simulink model "roll_model_TRUCKSIM_18DOF_REVISED"  (R2023b)
settings: Solver=FixedStepAuto  StartTime=0.0  StopTime=20  FixedStep=0.0005  RelTol=1e-3
StopFcn:
  | save_dataset_18state;
libraries: Solver_SF x1
(part 3 of 5)

== matlab function roll_model_TRUCKSIM_18DOF_REVISED/Subsystem2/MATLAB Function ==
  data: t input; ref12 output; scenario_id input; speed_case input; road_condition input; gamma_ref_prev input; hitch_diag output
function [ref12,hitch_diag] = fcn(t,scenario_id,speed_case,road_condition,gamma_ref_prev)
%#codegen
% =========================================================================
% BLOCK 1 - ROAD CONDITION + REFERENCE + ONLINE OPTIMAL HITCH ANGLE
%
% No CasADi. The hitch/articulation reference is obtained by a fixed-size
% 1-D grid optimization suitable for a Simulink MATLAB Function block.
%
% Inputs
%   t               scalar time [s]
%   scenario_id     1 straight, 2 single LC, 3 DLC, 4 slalom
%                   5 true parametric figure-eight stress path
%                   6 aggressive sharp S-turn / rapid DLC
%                   7 moderate fixed-geometry DLC for TruckSim tracking tests
%                   8 sharp LEFT 90-degree turn; 9 sharp RIGHT 90-degree turn
%   speed_case      1 constant 40 km/h, 2 accel/hold/brake, 3 smooth 40->60
%                   For scenario 7: levels 1..5 = 50, 56, 62, 66, 70 km/h.
%                   For scenario 8/9: automatically overrides with
%                   friction-aware deceleration / curve / acceleration.
%   road_condition  1 dry, 2 wet, 3 snow, 4 ice
%   gamma_ref_prev  previous optimal articulation reference in TruckSim sign [rad]
%
% ref12 =
%   1  vx_ref       [m/s]
%   2  ax_ref       [m/s^2]
%   3  Y_ref        [m]
%   4  dY_ref       [m/s]
%   5  psi_ref      [rad]
%   6  rt_ref       [rad/s]
%   7  drt_ref      [rad/s^2]
%   8  gamma_ref    [rad]     optimized hitch/articulation angle
%   9  rs_ref       [rad/s]
%  10  drs_ref      [rad/s^2]
%  11  kappa_ref    [1/m]
%  12  mu_road      [-]
%
% hitch_diag =
%   1 gamma_kin     geometric hitch target (smoothed for 8/9) [rad]
%   2 gamma_ref     final feasible optimized articulation [rad]
%   3 rho_y_opt     approximate lateral-friction use at trailer [-]
%   4 J_opt         local hitch cost [-]
%
% SHARP 90-DEG TURN (8/9): EXACT 25 m quarter circle, 20 m entry/exit.
% XY geometry: straight along X -> quarter-circle -> vertical tangent.
% Last part has X_ref = Lentry + R EXACTLY, not a diagonal line.
% NOTE ref12 has no X_ref channel; a separate XY verification file is bundled.
% For the exact circle, curvature/yaw-rate have steps at the joins.
% Hitch uses a 22m smooth-in / 24m smooth-out QUINTIC profile (C2).
% Explicit spatial derivatives generate consistent trailer yaw references.
% For 8/9 the hitch profile is deterministic and does not rely on the
% external gamma_ref_prev Unit Delay; scenarios 1-7 use that feedback.
%
% The uploaded circular-curve OCP motivates the local cost: preserve
% road-following kinematics while penalizing articulation magnitude,
% hitch/lateral demand, and reference variation. This is a LOCAL online
% optimum, not the global CasADi OCP.
% =========================================================================

Ts = 0.01;
ref12 = zeros(12,1);
hitch_diag = zeros(4,1);

%% Road friction map
if road_condition < 1.5
    mu_road = 0.85;      % dry
elseif road_condition < 2.5
    mu_road = 0.60;      % wet
elseif road_condition < 3.5
    mu_road = 0.35;      % snow
else
    mu_road = 0.20;      % ice
end


%% SCENARIO 12 - RAMP-STEER / J-TURN (OPEN-LOOP ROLL VALIDATION)
% Test ONLY active roll moment; no lateral Y tracking reference.
% speed_case sets STEER AMPLITUDE (not speed):
%   1: 2 deg, 2: 4 deg, 3: 6 deg, 4: 8 deg (road-wheel angle).
% In TruckSim Procedure select fixed target speed 40 km/h for the
% baseline runs; do NOT keep the old SPEED_TARGET_EQUATION (40+1.5*X)/3.6.
% Block 2 overrides steering directly and keeps Fx_req = 0, so TruckSim's
% own constant-speed driver must hold vx. Keep its drive torque imports off.
% ref12 is still 12x1 and hitch_diag 4x1. These refs are NOT Y trajectories.
if scenario_id >= 11.5 && scenario_id < 12.5
    if road_condition < 1.5
        mu_road = 0.80;     % nominal baseline from TruckSim .par
    end
    ref12(1)  = 40.0/3.6;  % desired constant speed for diagnostic only
    ref12(2)  = 0.0;
    ref12(3)  = 0.0;       % not used by open-loop Block 2
    ref12(4)  = 0.0;
    ref12(5)  = 0.0;
    ref12(6)  = 0.0;
    ref12(7)  = 0.0;
    ref12(8)  = 0.0;
    ref12(9)  = 0.0;
    ref12(10) = 0.0;
    % Temporary reuse of curvature slot for requested ROAD-WHEEL steer
    % amplitude [rad]. Block 2 reads it only in scenario 12. This is
    % necessary because Block 2 has NO speed_case input port.
    steerLevelsDeg = [2.0,4.0,6.0,8.0];
    idxSteer = min(max(round(speed_case),1),4);
    ref12(11) = steerLevelsDeg(idxSteer)*pi/180.0;
    ref12(12) = mu_road;
    return;
end

%% SCENARIO 10 - RIGHT TURN R20, SMOOTH CURVATURE, LTR VALIDATION
% All references are time-consistent and share the SAME path arclength.
% x(5) in the reconstructed TruckSim state follows dgamma = rt-rs;
% therefore ref12(8) uses the SAME model sign (not -gamma).
if scenario_id >= 9.5 && scenario_id < 10.5
    if road_condition < 1.5
        mu_road = 0.80;  % TruckSim .par nominal MU_REF_X/Y = 0.80
    end
    [v0,a0,Y0,dY0,psi0,rt0,k0] = tight_right_reference(t,speed_case,mu_road);
    [~,~,~,~,~,rt1,~] = tight_right_reference(t+Ts,speed_case,mu_road);
    [~,~,~,~,~,rt2,~] = tight_right_reference(t+2*Ts,speed_case,mu_road);

    gam0 = tight_right_gamma(t,speed_case,mu_road);
    gam1 = tight_right_gamma(t+Ts,speed_case,mu_road);
    gam2 = tight_right_gamma(t+2*Ts,speed_case,mu_road);
    gamDot0 = (gam1-gam0)/Ts;
    gamDot1 = (gam2-gam1)/Ts;

    ref12(1)=v0;
    ref12(2)=a0;
    ref12(3)=Y0;
    ref12(4)=dY0;
    ref12(5)=psi0;
    ref12(6)=rt0;
    ref12(7)=clamp((rt1-rt0)/Ts,-0.8,0.8);
    ref12(8)=gam0;                    % gamma=psi_t-psi_s, SAME as x(5)
    ref12(9)=rt0-gamDot0;
    ref12(10)=clamp(ref12(7)-(gamDot1-gamDot0)/Ts,-1.0,1.0);
    ref12(11)=k0;
    ref12(12)=mu_road;
    hitch_diag(1)=gam0;
    hitch_diag(2)=gam0;
    hitch_diag(3)=v0*v0*abs(k0)/max(mu_road*9.81,0.1);
    hitch_diag(4)=0.0;
    return;
end

%% SCENARIO 11 - SEVERE DOUBLE LANE CHANGE (simulation-only)
% 0 -> +3.5 m -> 0, two 42 m transitions, 12 m gap.
% Same 12-channel interface as every existing scenario.
% Dry road based on TruckSim nominal mu=0.80. Do not use as a claimed
% ISO 3888-2 standardized track: it is a custom heavy-truck DLC stress test.
if scenario_id >= 10.5 && scenario_id < 11.5
    if road_condition < 1.5
        mu_road=0.80;
    end
    [v0,a0,Y0,dY0,psi0,rt0,k0] = severe_dlc_reference(t,speed_case,mu_road);
    [~,~,~,~,~,rt1,~] = severe_dlc_reference(t+Ts,speed_case,mu_road);

    g0 = severe_dlc_gamma(t,speed_case,mu_road);
    g1 = severe_dlc_gamma(t+Ts,speed_case,mu_road);
    g2 = severe_dlc_gamma(t+2.0*Ts,speed_case,mu_road);
    gd0=(g1-g0)/Ts;
    gd1=(g2-g1)/Ts;
    dr0=clamp((rt1-rt0)/Ts,-0.80,0.80);

    ref12(1)=v0;
    ref12(2)=a0;
    ref12(3)=Y0;
    ref12(4)=dY0;
    ref12(5)=psi0;
    ref12(6)=rt0;
    ref12(7)=dr0;
    ref12(8)=g0;            % x(5) = psi_tractor - psi_trailer
    ref12(9)=rt0-gd0;
    ref12(10)=clamp(dr0-(gd1-gd0)/Ts,-1.0,1.0);
    ref12(11)=k0;
    ref12(12)=mu_road;
    hitch_diag(1)=g0;
    hitch_diag(2)=g0;
    hitch_diag(3)=v0*v0*abs(k0)/max(mu_road*9.81,0.1);
    hitch_diag(4)=0.0;
    return;
end

%% Current and preview base references
[vx0,ax0,Y0,dY0,psi0,rt0,kappa0] = ...
    base_reference(t,scenario_id,speed_case,mu_road);
[vx1,~,~,~,~,rt1,kappa1] = ...
    base_reference(t+Ts,scenario_id,speed_case,mu_road);
[vx2,~,~,~,~,rt2,kappa2] = ...
    base_reference(t+2.0*Ts,scenario_id,speed_case,mu_road);

%% Friction-aware longitudinal acceleration reference limit
% Keep the path/speed scenario recognizable, but do not ask for an
% impossible longitudinal acceleration on a low-mu road.
ax_lim = 0.45*mu_road*9.81;
ax0 = clamp(ax0,-ax_lim,ax_lim);

%% Online optimized hitch/articulation reference
% IMPORTANT SIGN CONVENTION:
%   internal model / geometry : gamma_m = psi_t - psi_s
%   TruckSim signal           : gamma_TS = psi_s - psi_t = -gamma_m
% gamma_ref_prev comes from ref12(8), therefore it is in TruckSim sign.
gamma_prev_model = -gamma_ref_prev;

% Scenario 8/9: deterministic, C2-smooth geometry-based hitch profile.
% This removes sudden rectangular reference jumps even if the Unit Delay
% feeding gamma_ref_prev is not configured correctly. Scenarios 1-7 use
% their original 31-candidate online optimizer and feasibility filtering.
isSharp = (scenario_id >= 7.5 && scenario_id < 9.5);

if isSharp
    turnSign=1.0;
    if scenario_id >= 8.5
        turnSign=-1.0;
    end

    % The sharp-turn reference is generated from s(t), not from the previous
    % sample. It has smooth analytic first/second derivatives.
    [gamma0,gammaKin0,gammaDot0,gammaDDot0,rho0,J0] = ...
        sharp_hitch_profile(t,mu_road,turnSign);

    % Internal articulation convention: gamma = psi_t-psi_s,
    % gamma_dot = r_t-r_s. Keep trailer yaw refs kinematically consistent.
    rs0 = rt0-gammaDot0;

    % Exact quarter-circle has curvature STEPS at its entry/exit. Its true
    % drt_ref has impulses there; bound only the feedforward acceleration
    % used by the SMC controller, preserving exact psi_ref/rt_ref/kappa_ref.
    drt0=(rt1-rt0)/Ts;
    drt0=clamp(drt0,-0.80,0.80);
    drs0=drt0-gammaDDot0;

else
    % ---------------------------------------------------------------
    % SCENARIOS 1-7: LEGACY HITCH OPTIMIZATION AND GAINS
    % ---------------------------------------------------------------
    [gammaOpt0,gammaKin0,rho0,J0] = optimal_hitch_angle( ...
        vx0,rt0,kappa0,mu_road,gamma_prev_model,false);

    alphaHitch = 0.50;
    gammaAmpGain = 1.550;
    dGammaFromKinMax = 2.0*pi/180.0;
    gammaRateMax = 15.0*pi/180.0;
    gammaRefMax = 10.0*pi/180.0;

    gamma0 = feasible_hitch_reference( ...
        gammaOpt0,gammaKin0,gamma_prev_model, ...
        alphaHitch,gammaAmpGain,dGammaFromKinMax, ...
        gammaRateMax,gammaRefMax,Ts);

    [gammaOpt1,gammaKin1,~,~] = optimal_hitch_angle( ...
        vx1,rt1,kappa1,mu_road,gamma0,false);
    gamma1 = feasible_hitch_reference( ...
        gammaOpt1,gammaKin1,gamma0, ...
        alphaHitch,gammaAmpGain,dGammaFromKinMax, ...
        gammaRateMax,gammaRefMax,Ts);

    [gammaOpt2,gammaKin2,~,~] = optimal_hitch_angle( ...
        vx2,rt2,kappa2,mu_road,gamma1,false);
    gamma2 = feasible_hitch_reference( ...
        gammaOpt2,gammaKin2,gamma1, ...
        alphaHitch,gammaAmpGain,dGammaFromKinMax, ...
        gammaRateMax,gammaRefMax,Ts);

    dgamma0 = wrap_pi(gamma1-gamma0)/Ts;
    dgamma1 = wrap_pi(gamma2-gamma1)/Ts;
    rs0 = rt0-dgamma0;
    rs1 = rt1-dgamma1;
    drt0 = (rt1-rt0)/Ts;
    drs0 = (rs1-rs0)/Ts;
end

%% Pack outputs
ref12(1)=vx0;
ref12(2)=ax0;
ref12(3)=Y0;
ref12(4)=dY0;
ref12(5)=psi0;
ref12(6)=rt0;
ref12(7)=drt0;
ref12(8)=-gamma0;  % TruckSim hitch sign: psi_s-psi_t
ref12(9)=rs0;
ref12(10)=drs0;
ref12(11)=kappa0;
ref12(12)=mu_road;

hitch_diag(1)=-gammaKin0; % TruckSim sign for direct comparison with x(5)
hitch_diag(2)=-gamma0;    % FINAL feasible reference, TruckSim sign
hitch_diag(3)=rho0;
hitch_diag(4)=J0;

end


% =========================================================================
% BASE ROAD / MANEUVER REFERENCE
% =========================================================================
function [vx_ref,ax_ref,Y_ref,dY_ref,psi_ref,rt_ref,kappa_ref] = ...
    base_reference(t,scenario_id,speed_case,mu_road)
%#codegen

v0 = 40.0/3.6;

% EXACT QUARTER-CIRCLE 8/9.
% For this stress test, speed_case is overridden by friction-aware speed.
if scenario_id >= 7.5 && scenario_id < 9.5
    turnDirection = 1.0;
    if scenario_id >= 8.5
        turnDirection = -1.0;
    end
    [vx_ref,ax_ref,Y_ref,dY_ref,psi_ref,rt_ref,kappa_ref] = ...
        sharp_turn_reference(t,mu_road,turnDirection);
    return;
end

% Fixed-geometry DLC. The other maneuvers retain their own speed profiles.
if scenario_id >= 6.5 && scenario_id < 7.5
    [vx_ref,ax_ref,Y_ref,dY_ref,psi_ref,rt_ref,kappa_ref] = ...
        dlc_load_transfer_reference(t,speed_case,mu_road);
    return;
end

%% Speed scenario used by scenarios 1-4 and 6
if speed_case < 1.5
    vx_base = v0;
    ax_base = 0.0;
elseif speed_case < 2.5
    if t < 5.0
        ax_base = 0.40;
        vx_base = v0+0.40*t;
    elseif t < 10.0
        ax_base = 0.0;
        vx_base = v0+2.0;
    elseif t < 16.0
        ax_base = -0.60;
        vx_base = v0+2.0-0.60*(t-10.0);
    else
        ax_base = 0.0;
        vx_base = v0+2.0-3.60;
    end
else
    v1=60.0/3.6;
    tc=8.0;
    wv=2.0;
    z=(t-tc)/wv;
    th=tanh(z);
    q=1.0-th*th;
    vx_base=v0+0.5*(v1-v0)*(1.0+th);
    ax_base=0.5*(v1-v0)*q/wv;
end

%% ========================================================================
% SCENARIO 5: TRUE PARAMETRIC FIGURE-EIGHT
%
% Gerono lemniscate:
%   X = A sin(theta)
%   Y = Yc + B sin(theta) cos(theta)
%
% theta starts at -pi/4 so the path begins with Y=0 and dY=0.
% A full loop is completed in T8 seconds. The speed reference is the tangent
% speed of the parametric curve, so speed_case is intentionally ignored for
% scenario 5.
%
% NOTE: Block 2 currently tracks Y, psi and yaw rate, not X_ref. Therefore
% this is a genuine geometric figure-eight reference for heading/curvature/Y,
% but exact XY closure would require adding X_ref or path-coordinate tracking.
% ========================================================================
if scenario_id >= 4.5 && scenario_id < 5.5
    t0 = 2.0;
    % Feasible low-speed figure-eight. The previous A=20,B=8,T=8 case
    % required about 45-50 deg road-wheel steering at the tightest point,
    % which is impossible under the high-speed 5-deg steering limit.
    T8 = 18.0;
    A8 = 14.0;   % longitudinal half-size [m]
    B8 = 16.0;   % lateral scale, Y approximately 0..16 m
    Yc = B8/2.0;
    om = 2.0*pi/T8;

    if t < t0 || t > t0+T8
        vx_ref = v0;
        ax_ref = 0.0;
        Y_ref = 0.0;
        dY_ref = 0.0;
        psi_ref = 0.0;
        rt_ref = 0.0;
        kappa_ref = 0.0;
        return;
    end

    theta = -pi/4.0 + om*(t-t0);

    xd  = A8*om*cos(theta);
    yd  = B8*om*cos(2.0*theta);
    xdd = -A8*om*om*sin(theta);
    ydd = -2.0*B8*om*om*sin(2.0*theta);

    Y_ref  = Yc + B8*sin(theta)*cos(theta);
    dY_ref = yd;

    vPath = sqrt(xd*xd+yd*yd);
    vx_ref = max(vPath,3.0);
    ax_ref = (xd*xdd+yd*ydd)/max(vPath,1.0e-6);

    psi_ref = atan2(yd,xd);
    rt_ref = (xd*ydd-yd*xdd)/max(xd*xd+yd*yd,1.0e-6);
    kappa_ref = (xd*ydd-yd*xdd) / ...
        max((xd*xd+yd*yd)^(1.5),1.0e-6);
    return;
end

%% Default speed reference for all remaining scenarios
vx_ref = vx_base;
ax_ref = ax_base;

%% Lateral road/maneuver scenario
if scenario_id < 1.5
    % 1: Straight
    Y_ref=0.0;
    dY_ref=0.0;
    ddY_ref=0.0;

elseif scenario_id < 2.5
    % 2: Single lane change 0 -> 3.5 m
    W=3.5;
    tc=8.0;
    wy=1.2;
    z=(t-tc)/wy;
    th=tanh(z);
    q=1.0-th*th;
    Y_ref=0.5*W*(1.0+th);
    dY_ref=0.5*W*q/wy;
    ddY_ref=-W*th*q/(wy*wy);

elseif scenario_id < 3.5
    % 3: Standard double lane change 0 -> 3.5 -> 0 m
    A=1.75;
    t1=6.5;
    t2=14.75;
    w=1.0;
    z1=(t-t1)/w;
    z2=(t-t2)/w;
    th1=tanh(z1);
    th2=tanh(z2);
    q1=1.0-th1*th1;
    q2=1.0-th2*th2;
    Y_ref=A*(th1-th2);
    dY_ref=(A/w)*(q1-q2);
    ddY_ref=(A/(w*w))*(-2.0*th1*q1+2.0*th2*q2);

elseif scenario_id < 4.5
    % 4: Continuous slalom
    A=1.5;
    freq=0.10;
    om=2.0*pi*freq;
    Y_ref=A*sin(om*t);
    dY_ref=A*om*cos(om*t);
    ddY_ref=-A*om*om*sin(om*t);

else
    % 6: AGGRESSIVE SHARP S-TURN / RAPID DLC
    % Larger lateral excursion + smaller transition width than scenario 3.
    % This intentionally stresses road-mu, ESO, hitch and roll control.
    A=2.25;       % peak lateral displacement about 4.5 m
    t1=5.5;
    t2=10.0;
    w=0.50;       % smaller -> sharper
    z1=(t-t1)/w;
    z2=(t-t2)/w;
    th1=tanh(z1);
    th2=tanh(z2);
    q1=1.0-th1*th1;
    q2=1.0-th2*th2;
    Y_ref=A*(th1-th2);
    dY_ref=(A/w)*(q1-q2);
    ddY_ref=(A/(w*w))*(-2.0*th1*q1+2.0*th2*q2);
end

vx_safe=max(abs(vx_ref),1.0);
psi_ref=atan2(dY_ref,vx_safe);
rt_ref=(vx_safe*ddY_ref-dY_ref*ax_ref) / ...
    max(vx_safe*vx_safe+dY_ref*dY_ref,1.0e-6);
kappa_ref=rt_ref/max(abs(vx_ref),1.0);

end


% =========================================================================
% SCENARIO 7 - MODERATE FIXED-GEOMETRY DLC
% =========================================================================
function [vx_ref,ax_ref,Y_ref,dY_ref,psi_ref,rt_ref,kappa_ref] = ...
    dlc_load_transfer_reference(t,speed_case,mu)
%#codegen
% Use a dry TruckSim road for the speed sweep. All levels share one path.
speedLevelsKmh = [50.0,56.0,62.0,66.0,70.0];
speedLevel = clamp(round(speed_case),1,5);
v0 = 40.0/3.6;
vDLC = speedLevelsKmh(speedLevel)/3.6;

% Accelerate on the straight with continuous acceleration and jerk.
settleTime = 2.5;
peakAx = min(1.35,0.45*mu*9.81);
rampTime = max(3.0,1.875*(vDLC-v0)/peakAx);
fraction = clamp(t/rampTime,0.0,1.0);
speedBlend = fraction^3*(10.0-fraction*(15.0-6.0*fraction));
vx_ref = v0+(vDLC-v0)*speedBlend;
ax_ref = (vDLC-v0)*30.0*fraction^2*(1.0-fraction)^2/rampTime;

% Arc length from the start of the first lane change. The vehicle is already
% at the target speed during both lane changes and the short straight between them.
laneShift = 3.5;
changeLength = 50.0;  % arc length of each lane change [m]
gapLength = 10.0;
s = vDLC*(t-rampTime-settleTime);

[outShape,outSlope,outBend] = dlc_lane_transition(s/changeLength);
[backShape,backSlope,backBend] = ...
    dlc_lane_transition((s-changeLength-gapLength)/changeLength);

Y_ref = laneShift*(outShape-backShape);
dY_ds = laneShift*(outSlope-backSlope)/changeLength;
d2Y_ds2 = laneShift*(outBend-backBend)/changeLength^2;

% s is path arc length: dY/ds = sin(psi) and dX/ds = cos(psi) > 0.
% Heading, yaw rate and curvature follow from the same road geometry.
dY_ref = vx_ref*dY_ds;
psi_ref = asin(dY_ds);
kappa_ref = d2Y_ds2/sqrt(1.0-dY_ds^2);
rt_ref = vx_ref*kappa_ref;

end


function [shape,slope,bend] = dlc_lane_transition(normalizedDistance)
%#codegen
% Unit 0-to-1 transition with its first three derivatives zero at each join.
u = clamp(normalizedDistance,0.0,1.0);
remaining = 1.0-u;
shape = u^4*(35.0-u*(84.0-u*(70.0-20.0*u)));
slope = 140.0*u^3*remaining^3;
bend = 420.0*u^2*remaining^2*(1.0-2.0*u);
end


% =========================================================================
% SCENARIOS 8/9 - EXACT QUARTER CIRCLE (20 m + R=25 m + vertical exit)
% =========================================================================
function [vx_ref,ax_ref,Y_ref,dY_ref,psi_ref,rt_ref,kappa_ref] = ...
    sharp_turn_reference(t,mu,turnDirection)
%#codegen
% Global coordinates: entering along +X, exiting along +/-Y.
% Path speed and distance share one analytic time profile.
[vx_ref,ax_ref,sProgress] = sharp_speed_progress(t,mu);
[Xtmp,Y_ref,psi_ref,kappa_ref] = ...
    exact_quarter_geometry(sProgress,turnDirection); %#ok<ASGLU>

dY_ref = vx_ref*sin(psi_ref);  % global lateral velocity [m/s]
rt_ref = vx_ref*kappa_ref;     % yaw rate [rad/s]
end


% =========================================================================
% FRICTION-AWARE SPEED + DISTANCE (SCENARIO 8/9 ONLY)
% =========================================================================
function [vx_ref,ax_ref,sProgress] = sharp_speed_progress(t,mu)
%#codegen
% Common analytical s(t) eliminates gaps/overlap between path segments.
% Smooth deceleration over 20m, constant curve speed, smooth acceleration
% over the next 20m. Curve speed is always < 8m/s so Block 2 permits 12 deg
% of road-wheel steering, enough for approx atan(3.49/25)=7.95 deg.
Rturn = 25.0;
Lentry = 25.0;
Lexit = 37.0;
SturnEnd = Lentry+0.5*pi*Rturn;
muSafe = clamp(mu,0.15,1.20);

vCurve = sqrt(0.28*muSafe*9.81*Rturn);
vCurve = clamp(vCurve,2.5,7.2);

% From peak smoothstep acceleration 0.75*(vEntry^2-vCurve^2)/Lentry.
aLongSafe = 0.40*muSafe*9.81;
vEntryLim = sqrt(vCurve*vCurve+(4.0/3.0)*aLongSafe*Lentry);
vEntry = min(40.0/3.6,vEntryLim);
vExit = vEntry;

Tentry = 2.0*Lentry/max(vEntry+vCurve,1.0e-6);
Tcurve = (0.5*pi*Rturn)/max(vCurve,1.0e-6);
Texit = 2.0*Lexit/max(vCurve+vExit,1.0e-6);
tq = max(t,0.0);

if tq < Tentry
    z=clamp(tq/Tentry,0.0,1.0);
    h=3.0*z*z-2.0*z*z*z;
    hInt=z*z*z-0.5*z*z*z*z;
    vx_ref=vEntry+(vCurve-vEntry)*h;
    ax_ref=(vCurve-vEntry)*(6.0*z-6.0*z*z)/Tentry;
    sProgress=vEntry*tq+(vCurve-vEntry)*Tentry*hInt;

elseif tq < Tentry+Tcurve
    dt=tq-Tentry;
    vx_ref=vCurve;
    ax_ref=0.0;
    sProgress=Lentry+vCurve*dt;

elseif tq < Tentry+Tcurve+Texit
    dt=tq-Tentry-Tcurve;
    z=clamp(dt/Texit,0.0,1.0);
    h=3.0*z*z-2.0*z*z*z;
    hInt=z*z*z-0.5*z*z*z*z;
    vx_ref=vCurve+(vExit-vCurve)*h;
    ax_ref=(vExit-vCurve)*(6.0*z-6.0*z*z)/Texit;
    sProgress=SturnEnd+vCurve*dt+(vExit-vCurve)*Texit*hInt;

else
    dt=tq-Tentry-Tcurve-Texit;
    vx_ref=vExit;
    ax_ref=0.0;
    sProgress=SturnEnd+Lexit+vExit*dt;
end
end


% =========================================================================
% EXACT XY GEOMETRY: STRAIGHT -> QUARTER CIRCLE -> VERTICAL TANGENT
% =========================================================================
function [X_ref,Y_ref,psi_ref,kappa_ref] = ...
    exact_quarter_geometry(sProgress,turnDirection)
%#codegen
Rturn=25.0;
Lentry=20.0;
turnAngle=0.5*pi;
SturnEnd=Lentry+Rturn*turnAngle;
s=max(sProgress,0.0);

if s<=Lentry
    X_ref=s;
    Y_ref=0.0;
    psi_ref=0.0;
    kappa_ref=0.0;

elseif s<SturnEnd
    theta=(s-Lentry)/Rturn;
    X_ref=Lentry+Rturn*sin(theta);
    Y_ref=turnDirection*Rturn*(1.0-cos(theta));
    psi_ref=turnDirection*theta;
    kappa_ref=turnDirection/Rturn;

else
    sOut=s-SturnEnd;
    X_ref=Lentry+Rturn;                      % EXACTLY 45 m, always
    Y_ref=turnDirection*(Rturn+sOut);        % straight UP or DOWN
    psi_ref=turnDirection*turnAngle;         % EXACTLY +/- pi/2
    kappa_ref=0.0;
end
end


% =========================================================================
% SCENARIO 8/9 - SMOOTH 90-DEG HITCH REFERENCE (NO RECTANGULAR STEPS)
% =========================================================================
function [gammaModel,gammaKinShape,gammaDot,gammaDDot,rho,J] = ...
    sharp_hitch_profile(t,mu,turnDirection)
%#codegen
% The XY path remains EXACT: straight, 90-degree R25 circular arc, vertical
% exit. Only hitch target is shaped in DISTANCE using a quintic C2 window.
%
% The target is DETERMINISTIC in time. No hidden persistent states and no
% dependence on gamma_ref_prev for scenarios 8/9. This guarantees that
% gamma_ref, rs_ref and drs_ref describe the same continuous trajectory.
%
% Distance windows (modifiable):
%   entry ramp starts 6m BEFORE arc, ends 16m INSIDE arc  (22m total)
%   exit  ramp starts 11m BEFORE arc end, ends 13m AFTER (24m total)
% Steady hitch magnitude is near 10.05deg for R=25m; TruckSim sign is
% applied in the main function when output ref12(8)=-gammaModel.

Rturn=25.0;
Lentry=20.0;
S3=Lentry+0.5*pi*Rturn;

% >>> TWO PRIMARY HITCH SMOOTHNESS SETTINGS <<<
sInStart=Lentry-6.0;
sInEnd=Lentry+16.0;
sOutStart=S3-11.0;
sOutEnd=S3+13.0;

[vx,ax,s]=sharp_speed_progress(t,mu);

% Kinematic articulation seed + bounded LOCAL 31-point optimizer.
% Steady-state value is calculated once mathematically for this R and mu.
kappaArc=turnDirection/Rturn;
Lwt=1.444869792;
Lrs=8.500;
a=Lwt*kappaArc;
arg=clamp(Lrs*kappaArc/sqrt(1.0+a*a),-0.98,0.98);
gammaKinSS=atan(a)+asin(arg);

muSafe=clamp(mu,0.15,1.20);
vCurve=clamp(sqrt(0.28*muSafe*9.81*Rturn),2.5,7.2);
[gammaOptSS,~,rhoSS,J] = optimal_hitch_angle( ...
    vCurve,vCurve*kappaArc,kappaArc,mu,gammaKinSS,true);

% Geometry remains the dominant term. Optimizer may move the steady-state
% seed by at most 0.5deg and only 15% of that correction is included.
deltaOpt=clamp(gammaOptSS-gammaKinSS, ...
              -0.5*pi/180.0,0.5*pi/180.0);
gammaSS=gammaKinSS+0.15*deltaOpt;
gammaSS=clamp(gammaSS,-12.0*pi/180.0,12.0*pi/180.0);

% Smoothstep5 guarantees W, W_s and W_ss connect without jumps.
[win,winS,winSS] = quintic_ramp(s,sInStart,sInEnd);
[wout,woutS,woutSS] = quintic_ramp(s,sOutStart,sOutEnd);

% W(s) rises 0->1, stays near 1 over arc, falls 1->0.
W=win*(1.0-wout);
Ws=winS*(1.0-wout)-win*woutS;
Wss=winSS*(1.0-wout)-2.0*winS*woutS-win*woutSS;

gammaModel=gammaSS*W;
gammaKinShape=gammaKinSS*W;

% Time derivatives from s_dot=v and s_ddot=ax.
gammaDot=gammaSS*Ws*vx;
gammaDDot=gammaSS*(Wss*vx*vx+Ws*ax);

% Diagnostics are estimates, NOT measured TruckSim tire loads.
rho=rhoSS*W;
end


function [h,hs,hss]=quintic_ramp(s,s0,s1)
%#codegen
% h = 10 z^3 - 15 z^4 + 6 z^5, z=(s-s0)/(s1-s0).
% Derivatives are with respect to spatial path coordinate s [m].
L=max(s1-s0,1.0e-6);
z=(s-s0)/L;
if z<=0.0
    h=0.0; hs=0.0; hss=0.0;
elseif z>=1.0
    h=1.0; hs=0.0; hss=0.0;
else
    h=z*z*z*(10.0+z*(-15.0+6.0*z));
    hs=30.0*z*z*(1.0-z)*(1.0-z)/L;
    hss=60.0*z*(1.0-z)*(1.0-2.0*z)/(L*L);
end
end


% =========================================================================
% LOCAL OPTIMAL HITCH / ARTICULATION ANGLE
% =========================================================================
function [gammaOpt,gammaKin,rhoYOpt,Jbest] = ...
    optimal_hitch_angle(vx,rt,kappa,mu,gammaPrev,isSharp)
%#codegen

% Geometry must match vehicle_18dof_full_roll.m
Lwt = 1.444869792;   % tractor CG -> fifth wheel
Lrs = 8.500;   % fifth wheel -> trailer axle

gammaMax = 35.0*pi/180.0;

% Exact no-slip steady-turn geometric seed:
% sin(gamma)-Lwt*kappa*cos(gamma)-Lrs*kappa = 0
% => gamma = atan(Lwt*kappa) + asin(Lrs*kappa/sqrt(1+(Lwt*kappa)^2))
a = Lwt*kappa;
R = sqrt(1.0+a*a);
arg = clamp(Lrs*kappa/max(R,1.0e-8),-0.98,0.98);
gammaKin = atan(a)+asin(arg);
gammaKin = clamp(gammaKin,-gammaMax,gammaMax);

% Search locally around the geometric seed. 31 fixed candidates keeps the
% block code-generation friendly and deterministic.
searchHalf = 10.0*pi/180.0;
N = 31;

% ORIGINAL hitch optimization weights.
wKin    = 35.0;
wGamma  = 1.0;
wSmooth = 4.0;
wFric   = 6.0;
wHitch  = 1.5;

if isSharp
    % Sharp turn: enforce geometry more strongly and avoid lagging behind
    % the geometric articulation by penalizing the previous angle too much.
    % Still a fixed-size LOCAL grid optimizer, not a global OCP solution.
    searchHalf = 4.0*pi/180.0;
    wKin    = 80.0;
    wGamma  = 0.50;
    wSmooth = 0.30;
    wFric   = 8.0;
    wHitch  = 1.0;
end

Jbest = 1.0e30;
gammaOpt = gammaKin;
rhoYOpt = 0.0;

vSafe=max(abs(vx),0.5);
muG=max(mu*9.81,0.25);
rtScale=max(abs(rt),0.05);

gammaStepScale = 5.0*pi/180.0;

for i=1:N
    s=(i-1)/(N-1);
    gcand=gammaKin-searchHalf+2.0*searchHalf*s;
    gcand=clamp(gcand,-gammaMax,gammaMax);

    % Trailer yaw rate implied by fifth-wheel/trailer-axle no-slip geometry:
    % V_y,h^s - Lrs*r_s = 0
    rsKin=(vSafe*sin(gcand)-Lwt*rt*cos(gcand))/Lrs;

    eKin=(rsKin-rt)/rtScale;
    eGamma=gcand/gammaMax;
    eSmooth=wrap_pi(gcand-gammaPrev)/gammaStepScale;

    ayTrailer=vSafe*rsKin;
    rhoY=abs(ayTrailer)/muG;
    excess=max(rhoY-0.65,0.0);

    % Normalized hitch-force proxy based on trailer lateral acceleration.
    hitchProxy=abs(ayTrailer)/muG;

    J = wKin*eKin*eKin ...
        +wGamma*eGamma*eGamma ...
        +wSmooth*eSmooth*eSmooth ...
        +wFric*excess*excess ...
        +wHitch*hitchProxy*hitchProxy;

    if J<Jbest
        Jbest=J;
        gammaOpt=gcand;
        rhoYOpt=rhoY;
    end
end

% gammaOpt is intentionally returned as the RAW local optimum.
% Feasibility and rate limiting are applied outside this function so the
% final reference can be constrained relative to gammaKin.

end


function gammaRef=feasible_hitch_reference( ...
    gammaOpt,gammaKin,gammaPrev, ...
    alphaHitch,gammaAmpGain,dGammaMax, ...
    gammaRateMax,gammaRefMax,Ts)
%#codegen

%% Optimizer correction around geometric hitch angle
dGammaOpt = wrap_pi(gammaOpt-gammaKin);

dGammaOpt = clamp( ...
    dGammaOpt, ...
   -dGammaMax, ...
    dGammaMax);

%% Blend optimized correction
gammaBase = gammaKin ...
          + alphaHitch*dGammaOpt;

%% ---------------------------------------------------------------
% HITCH REFERENCE AMPLITUDE SHAPING
%
% This is the variable that DIRECTLY changes gamma_ref amplitude.
% gammaAmpGain > 1 -> larger reference
% gammaAmpGain < 1 -> smaller reference
% ---------------------------------------------------------------

gammaTarget = gammaAmpGain*gammaBase;

%% Absolute safety limit
gammaTarget = clamp( ...
    gammaTarget, ...
   -gammaRefMax, ...
    gammaRefMax);

%% Reference slew limit
gammaRef = rate_limit( ...
    gammaTarget, ...
    gammaPrev, ...
    gammaRateMax*Ts);

end


function y=rate_limit(target,previous,max_step)
%#codegen
d=wrap_pi(target-previous);
if d>max_step
    d=max_step;
elseif d<-max_step
    d=-max_step;
end
y=wrap_pi(previous+d);
end

function y=clamp(x,lo,hi)
%#codegen
if x>hi
    y=hi;
elseif x<lo
    y=lo;
else
    y=x;
end
end

function a=wrap_pi(a)
%#codegen
a=atan2(sin(a),cos(a));
end


% ========================================================================
% NEW SCENARIO 10 -- RIGHT-TURN LTR TEST
% 40m straight approach; R=20m, 90deg right turn; 35m straight exit.
% Curvature is quintic-ramped over 8m at each end of the circular arc.
% Time-varying speed is C1 and the XY path is continuous with C2 heading.
% This is deliberately a feasible closed-loop reference, not a fixed
% steering step; low speed increases the chance of successful tracking.
% ========================================================================
function [v,ax,Y,dY,psi,rt,kappa] = tight_right_reference(t,speed_case,mu)
%#codegen
[v,ax,s]=tight_right_speed(t,speed_case,mu);
[~,Y,psi,kappa]=tight_right_geometry(s);
dY=v*sin(psi);
rt=v*kappa;
end

function [v,ax,s] = tight_right_speed(t,speed_case,mu)
%#codegen
R=20.0;
Lentry=40.0;
Lramp=8.0;
Lcurve=0.5*pi*R+Lramp;
Lexit=35.0;
v0=12.0;          % matches default integrator initial vx
vlevel=[6.6,7.2,7.8,8.2];  % road curve speeds (m/s), speed_case=1..4
idx=int32(min(max(round(speed_case),1),4));
vc_nom=vlevel(idx);
vc=min(vc_nom,sqrt(0.42*max(mu,0.15)*9.81*R));
vc=max(vc,3.0);
% Ensure entry braking remains attainable on the requested road.
% At low mu lower initial speed must also be set in TruckSim and x0.
Tentry=2*Lentry/max(v0+vc,1.0);
Tcurve=Lcurve/vc;
Texit=2*Lexit/max(v0+vc,1.0);
tt=max(t,0.0);
if tt<Tentry
    z=min(max(tt/Tentry,0.0),1.0);
    h=z*z*(3.0-2.0*z);
    ih=z*z*z-0.5*z*z*z*z;
    v=v0+(vc-v0)*h;
    ax=(vc-v0)*6.0*z*(1.0-z)/Tentry;
    s=v0*tt+(vc-v0)*Tentry*ih;
elseif tt<Tentry+Tcurve
    dt=tt-Tentry;
    v=vc;
    ax=0.0;
    s=Lentry+vc*dt;
elseif tt<Tentry+Tcurve+Texit
    dt=tt-Tentry-Tcurve;
    z=min(max(dt/Texit,0.0),1.0);
    h=z*z*(3.0-2.0*z);
    ih=z*z*z-0.5*z*z*z*z;
    v=vc+(v0-vc)*h;
    ax=(v0-vc)*6.0*z*(1.0-z)/Texit;
    s=Lentry+Lcurve+vc*dt+(v0-vc)*Texit*ih;
else
    dt=tt-Tentry-Tcurve-Texit;
    v=v0;
    ax=0.0;
    s=Lentry+Lcurve+Lexit+v0*dt;
end
end

function [X,Y,psi,kappa]=tight_right_geometry(s)
%#codegen
Lentry=40.0;
R=20.0;
Lramp=8.0;
Lflat=0.5*pi*R-Lramp;
Lcurve=Lflat+2.0*Lramp;
ss=max(s,0.0);
if ss<=Lentry
    X=ss;
    Y=0.0;
    psi=0.0;
    kappa=0.0;
    return;
end
u=min(ss-Lentry,Lcurve);
[psi,kappa]=tight_heading_curvature(u);
% Fixed-size Simpson quadrature: accurate, no persistent-state drift or
% unknown-size data, supports MATLAB Function Coder.
N=48;
dh=u/N;
ix=0.0;iy=0.0;
for j=0:N
    sj=dh*j;
    [psj,~]=tight_heading_curvature(sj);
    if j==0 || j==N
        w=1.0;
    elseif mod(j,2)==0
        w=2.0;
    else
        w=4.0;
    end
    ix=ix+w*cos(psj);
    iy=iy+w*sin(psj);
end
X=Lentry+dh*ix/3.0;
Y=dh*iy/3.0;
if ss>Lentry+Lcurve
    extra=ss-(Lentry+Lcurve);
    psi=-0.5*pi;
    kappa=0.0;
    Y=Y-extra;
end
end

function [psi,kappa]=tight_heading_curvature(u)
%#codegen
R=20.0;
Lr=8.0;
Lc=0.5*pi*R-Lr;
Lend=2.0*Lr+Lc;
a=min(max(u,0.0),Lend);
if a<Lr
    z=a/Lr;
    h=z*z*z*(10.0-15.0*z+6.0*z*z);
    ih=2.5*z^4-3.0*z^5+z^6;
    theta=Lr*ih/R;
    k=h/R;
elseif a<Lr+Lc
    theta=(0.5*Lr+(a-Lr))/R;
    k=1.0/R;
else
    z=(a-Lr-Lc)/Lr;
    h=z*z*z*(10.0-15.0*z+6.0*z*z);
    ih=2.5*z^4-3.0*z^5+z^6;
    theta=(0.5*Lr+Lc+Lr*(z-ih))/R;
    k=(1.0-h)/R;
end
psi=-theta;
kappa=-k;
end

function gamma=tight_right_gamma(t,speed_case,mu)
%#codegen
% Articulation reference is generated by the no-slip kinematic model,
% integrated in spatial arclength.  It DOES NOT jump to the steady-state
% 29deg hitch angle when the tractor starts entering the curve.
%
% dgamma/ds = kappa - (sin(gamma)-Lwt*kappa*cos(gamma))/Lrs
% This ensures gammaDot=rt-rs and produces realistic trailer yaw-rate refs.
[~,~,s]=tight_right_speed(t,speed_case,mu);
N=128;                         % fixed-size loop for code generation
h=max(s,0.0)/N;
gamma=0.0;
for j=1:N
    sj=(j-1)*h;
    k1=tight_gamma_rhs(sj,gamma);
    k2=tight_gamma_rhs(sj+0.5*h,gamma+0.5*h*k1);
    k3=tight_gamma_rhs(sj+0.5*h,gamma+0.5*h*k2);
    k4=tight_gamma_rhs(sj+h,gamma+h*k3);
    gamma=gamma+(h/6.0)*(k1+2.0*k2+2.0*k3+k4);
end
gamma=clamp(gamma,-0.60,0.60);  % hard articulation reference bound
end

function dgamma_ds=tight_gamma_rhs(s,gamma)
%#codegen
[~,kappa]=tight_heading_curvature(s-40.0);
Lwt=1.444869792;
Lrs=8.50;
dgamma_ds=kappa-(sin(gamma)-Lwt*kappa*cos(gamma))/Lrs;
end



% =========================================================================
% SCENARIO 11: TRACKABLE DLC - GEOMETRICALLY CONSISTENT PATH REFERENCE
% s is path arc length, not world-X. Lateral derivative dY/ds=sin(psi).
% Trailer hitch reference is causally smoothed to avoid an instantaneous
% steady-turn articulation command at each yaw reversal.
% =========================================================================
function [v,ax,Y,dY,psi,rt,kappa] = severe_dlc_reference(t,speed_case,mu)
%#codegen
laneShift=3.50;   % m, 1 lane change
Lchange=42.0;   % m, each transition (42 m)
Lgap=12.0;        % m, straight connector
Tacc=5.0;         % s, smooth acceleration/deceleration first
Tsettle=0.8;      % s, straight before the first lateral movement
vStart=12.0;      % m/s, MUST match initial TruckSim and plant

vLevels=[13.0,14.5,16.0,17.5]; % speed_case 1..4 (m/s)
icase=min(max(round(speed_case),1),4);
vRequested=vLevels(icase);

% The closed-loop tracking test is invalid when tire friction is exceeded.
% For 7th-order lateral profile, maximum |d2(shape)/du2| = 7.513189.
kappaBound=laneShift/(Lchange*Lchange)*7.513189 / ...
    sqrt(1.0-(2.1875*laneShift/Lchange)^2);
vFric=sqrt(0.94*max(mu,0.20)*9.81/max(kappaBound,1.0e-6));
vCurve=min(vRequested,vFric);

if t<=0.0
    v=vStart;
    ax=0.0;
elseif t<Tacc
    u=t/Tacc;
    z=u*u*u*(10.0+u*(-15.0+6.0*u));
    zp=30.0*u*u*(1.0-u)*(1.0-u)/Tacc;
    v=vStart+(vCurve-vStart)*z;
    ax=(vCurve-vStart)*zp;
else
    v=vCurve;
    ax=0.0;
end

s=max(t-(Tacc+Tsettle),0.0)*vCurve;

[sh1,dsh1,ddsh1]=severe_dlc_shape(s/Lchange);
[sh2,dsh2,ddsh2]=severe_dlc_shape((s-Lchange-Lgap)/Lchange);

Y=laneShift*(sh1-sh2);
Ys=laneShift*(dsh1-dsh2)/Lchange;
Yss=laneShift*(ddsh1-ddsh2)/(Lchange*Lchange);
Ys=max(min(Ys,0.95),-0.95);
psi=asin(Ys);
dY=v*Ys;
kappa=Yss/sqrt(max(1.0-Ys*Ys,0.05));
rt=v*kappa;
end

function [h,hp,hpp] = severe_dlc_shape(z)
%#codegen
u=max(0.0,min(z,1.0));
h=u^4*(35.0-u*(84.0-u*(70.0-20.0*u)));
hp=140.0*u^3*(1.0-u)^3;
hpp=420.0*u^2*(1.0-u)^2*(1.0-2.0*u);
end

function gamma=severe_dlc_gamma(t,speed_case,mu)
%#codegen
% Deterministic 1.2 s causal smoothing of geometric fifth-wheel angle.
% Avoid relying on the Unit Delay sample time for the new scenario.
Lh=1.444869792;  % tractor CG to fifth wheel [m]
Ls=8.500;        % hitch to trailer axle [m]
weightSum=0.0;
angleSum=0.0;
for j=0:12
    tau=0.10*j;
    [~,~,~,~,~,~,kap]=severe_dlc_reference(t-tau,speed_case,mu);
    u=Lh*kap;
    ss=sqrt(1.0+u*u);
    ga=atan(u)+asin(max(-0.98,min(0.98,Ls*kap/ss)));
    ga=max(-0.35,min(0.35,ga));
    w=exp(-tau/0.45);
    angleSum=angleSum+w*ga;
    weightSum=weightSum+w;
end
gamma=angleSum/max(weightSum,1.0e-9);
end
